simulink model "toa_wl00_sim"  (Simulink 9.0)
settings: Solver=FixedStepDiscrete  StartTime=0  StopTime=350  FixedStep=0.02  RelTol=1e-3  EnableMultiTasking=on
PreLoadFcn:
  | makefile_build_callback(bdroot,'toa_wl00.buildescription');
undefined symbols (not defined in the file or in its folder): TIME, timestep, WeighDebug_TOAarbitrated_payload, WeighDebug_TOAbucket_current_w_1, WeighDebug_TOAbucket_current_wei, WeighDebug_TOAcurrent_weight_nor, WeighDebug_TOAeef_imu_accelX, WeighDebug_TOAeef_imu_accelY, WeighDebug_TOAeef_imu_accelZ, WeighDebug_TOAerror_code_out, WeighDebug_TOAinvalidate_outputs, WeighDebug_TOAlift_angle, WeighDebug_TOAlift_he_pressure, WeighDebug_TOAlift_re_pressure, WeighDebug_TOAlift_valve_cmd, WeighDebug_TOApayload_norm_stdev, WeighDebug_TOApayload_send_to_CP, WeighDebug_TOApayload_status_sen, WeighDebug_TOApcs_weight_accurac, WeighDebug_TOAspill_rate_out, WeighDebug_TOAsteering_angle, WeighDebug_TOAtilt_extension, WeighDebug_TOAtilt_he_pressure, WeighDebug_TOAtilt_pressure_out, WeighDebug_TOAtilt_re_pressure, WeighDebug_TOAtilt_sensitivity_o, WeighDebug_TOAtilt_valve_cmd, WeighDebug_TOAtipoff_mode, WeighDebug_TOAtool_mass, WeighDebug_TOAtruck_start_weight, WeighDebug_TOAtruck_target_wt, WeighDebug_TOAweigh_status_out
libraries: simulink x30, lib_CATutils_Utilities_ApplyName_v2 x3, tip_assist_lib_support x1
settings Model: MinMaxOverflowLogging=MinMaxAndOverflow  Creator=gulamhs  LastModifiedBy=gulamhs  SimulationMode=accelerator
settings DataIOCC: ExternalInput=[t,u]  SaveCompleteFinalSimState=on  SaveFormat=StructureWithTime  SaveOutput=off  SignalLogging=off  DSMLogging=off  SaveTime=off
settings OptimizationCC: DefaultParameterBehavior=Inlined  InlineInvariantSignals=on  EnhancedBackFolding=on  StrengthReduction=on  BitfieldContainerType=uchar_T  PassReuseOutputArgsAs=Individual arguments  ExpressionDepthLimit=2147483647  EfficientFloat2IntCast=on
settings DebuggingCC: SignalInfNanChecking=warning  SignalRangeChecking=error  ReadBeforeWriteMsg=EnableAllAsError  WriteAfterWriteMsg=EnableAllAsError  WriteAfterReadMsg=EnableAllAsError  AlgebraicLoopMsg=error  ArtificialAlgebraicLoopMsg=error  SaveWithDisabledLinksMsg=error  SaveWithParameterizedLinksMsg=error  UnderspecifiedInitializationDetection=Simplified  MergeDetectMultiDrivingBlocksExec=error  BlockPriorityViolationMsg=error  SolverPrmCheckMsg=error  InheritedTsInSrcMsg=none  TasksWithSamePriorityMsg=error  SigSpecEnsureSampleTimeMsg=error  CheckMatrixSingularityMsg=error  IntegerOverflowMsg=error  ParameterUnderflowMsg=error  ParameterPrecisionLossMsg=none  FixptConstUnderflowMsg=error  FixptConstOverflowMsg=error  UnderSpecifiedDataTypeMsg=error  FcnCallInpInsideContextMsg=warning  UnconnectedInputMsg=error  UnconnectedOutputMsg=error  UnconnectedLineMsg=error  SFcnCompatibilityMsg=error  FrameProcessingCompatibilityMsg=warning  UniqueDataStoreMsg=error  BusObjectLabelMismatch=error  RootOutportRequireBusObject=error  AssertControl=DisableAll  ModelReferenceIOMsg=error  ModelReferenceVersionMismatchMessage=warning  ModelReferenceIOMismatchMessage=error  UnknownTsInhSupMsg=error  ModelReferenceDataLoggingMessage=error  StateNameClashWarn=warning  SimStateInterfaceChecksumMismatchMsg=error  StrictBusMsg=ErrorOnBusTreatedAsVector  BusNameAdapt=ErrorWithoutRepair  NonBusSignalsTreatedAsBus=error  SFInvalidInputDataAccessInChartInitDiag=error  SFNoUnconditionalDefaultTransitionDiag=error  SFTransitionOutsideNaturalParentDiag=error  SFUnreachableExecutionPathDiag=error  SFUndirectedBroadcastEventsDiag=error  SFExecutionAtInitializationDiag=warning  IntegerSaturationMsg=error
settings HardwareCC: ProdBitPerLong=64  ProdBitPerPointer=64  ProdBitPerSizeT=64  ProdBitPerPtrDiffT=64  ProdLargestAtomicInteger=Integer  ProdLargestAtomicFloat=Float  ProdIntDivRoundTo=Zero  ProdEndianess=LittleEndian  ProdWordSize=64  ProdHWDeviceType=Intel->x86-64 (Linux 64)
settings ModelReferenceCC: ParallelModelReferenceMATLABWorkerInit=Load Top Model  PropagateSignalLabelsOutOfModel=on
settings SFSimCC: SFSimEcho=off  SimGenImportedTypeDefs=on  MATLABDynamicMemAlloc=off
settings RTWCC: SystemTargetFile=cat_PkgArch.tlc  GenCodeOnly=on  GenerateMakefile=off  TemplateMakefile=cat_PkgArch_default_tmf  Description=R7a CAT Package Architecture Code Generation.  GenerateReport=on  RTWUseSimCustomCode=on  CodeProfilingSaveOptions=AllData  GenerateTraceReport=on  GenerateTraceReportSl=on  GenerateTraceReportSf=on  GenerateTraceReportEml=on  GenerateWebview=on  GenerateCodeMetricsReport=on  GenerateCodeReplacementReport=on
settings CodeAppCC: ForceParamTrailComments=on  IgnoreCustomStorageClasses=off  MaxIdLength=63  OperatorAnnotations=on  SimulinkDataObjDesc=on  SFDataObjDesc=on  MATLABFcnDesc=on  MangleLength=4  CustomSymbolStrType=$N$R$M  InsertBlockDesc=on  MATLABSourceComments=on  InternalIdentifier=Classic  ReqsInCode=on  UseSimReservedNames=on
settings STFCustomTargetCC: UtilityFuncGeneration=Shared location  MultiwordTypeDef=User defined  IncludeMdlTerminateFcn=off  CombineOutputUpdateFcns=on  SuppressErrorStatus=on  ERTCustomFileBanners=on  SupportAbsoluteTime=off  MultiInstanceERTCode=on  CodeInterfacePackaging=Reusable function  SupportComplex=off  SupportContinuousTime=off  SupportNonInlinedSFcns=off  RemoveResetFunc=on  SupportVariableSizeSignals=on  ParenthesesLevel=Maximum  MATLABClassNameForMDSCustomization=Simulink.SoftwareTarget.ERTCustomization  GRTInterface=off  GenerateSharedConstants=off  SystemTargetFile=cat_PkgArch.tlc
settings ERTTargetCC: UtilityFuncGeneration=Shared location  MultiwordTypeDef=User defined  MultiwordLength=2048  ParMdlRefBuildCompliant=off  CompOptLevelCompliant=off  ConcurrentExecutionCompliant=off  IncludeMdlTerminateFcn=off  SuppressErrorStatus=on  SupportAbsoluteTime=off  MultiInstanceERTCode=on  CodeInterfacePackaging=Reusable function  SupportComplex=off  SupportVariableSizeSignals=on  ParenthesesLevel=Maximum  ModelStepFunctionPrototypeControlCompliant=off  CPPClassGenCompliant=off  UseToolchainInfoCompliant=off  GenerateSharedConstants=off  MultiInstanceErrorCode=None  ERTSrcFileBannerTemplate=cat_code_template.cgt  ERTHdrFileBannerTemplate=cat_code_template.cgt  ERTDataSrcFileTemplate=cat_code_template.cgt  ERTDataHdrFileTemplate=cat_code_template.cgt  ERTCustomFileTemplate=cat_PkgArch_CFP.tlc  SuppressUnreachableDefaultCases=off  EnableUserReplacementTypes=on
settings MATStruct: int32=int32_t  int16=int16_t  int8=int8_t  uint32=uint32_t  uint16=uint16_t  uint8=uint8_t
settings CustomProperty: Value=Development
settings EnumStrPairs: String=Development
settings ConfigComp: CovMetricSettings=dwe  CovHtmlReporting=off  CovSaveCumulativeToWorkspaceVar=off  CovSaveSingleToWorkspaceVar=off  CovExternalEMLEnable=on

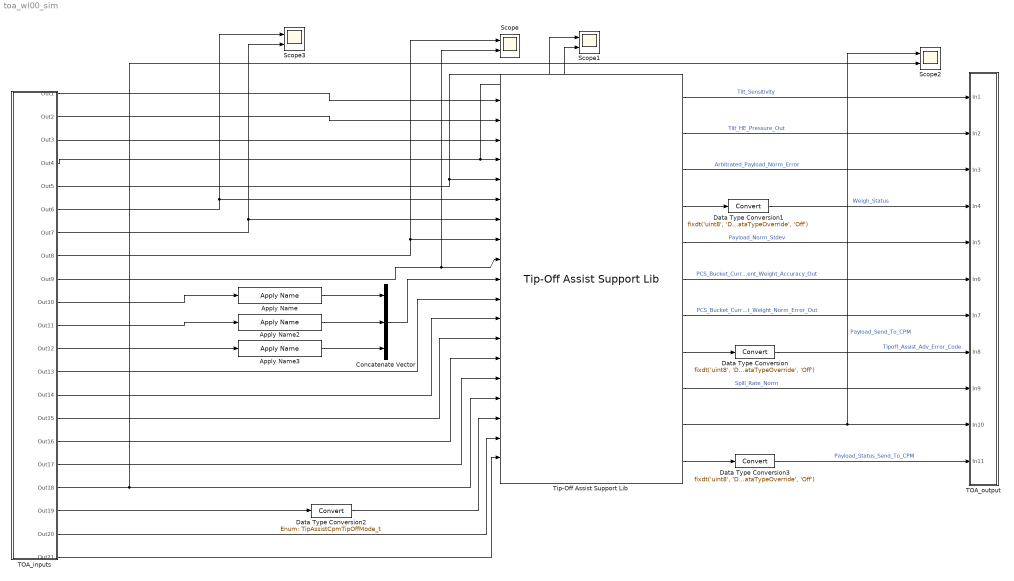
== system toa_wl00_sim ==
  Apply Name : lib_CATutils_Utilities_ApplyName_v2/Apply Name  sigLabel='toa_inImuAcclX'  enTst=true
  Apply Name2 : lib_CATutils_Utilities_ApplyName_v2/Apply Name  sigLabel='toa_inImuAcclY'  enTst=true
  Apply Name3 : lib_CATutils_Utilities_ApplyName_v2/Apply Name  sigLabel='toa_inImuAcclZ'  enTst=true
  Concatenate Vector : Concatenate  NumInputs=3  Mode=Multidimensional array
  Data Type Conversion : DataTypeConversion  OutMin=[0]  OutMax=[6]  OutDataTypeStr=fixdt('uint8', 'DataTypeOverride', 'Off')
  Data Type Conversion1 : DataTypeConversion  OutMin=[0]  OutMax=[5]  OutDataTypeStr=fixdt('uint8', 'DataTypeOverride', 'Off')
  Data Type Conversion2 : DataTypeConversion  OutDataTypeStr=Enum: TipAssistCpmTipOffMode_t
  Data Type Conversion3 : DataTypeConversion  OutMin=[0]  OutMax=[5]  OutDataTypeStr=fixdt('uint8', 'DataTypeOverride', 'Off')
  Scope{,1..3} (4 alike) : Scope  NumInputPorts=2
  "TOA_inputs " : Subsystem
  "TOA_output " : Subsystem
  Tip-Off Assist Support Lib : tip_assist_lib_support/Tip-Off Assist Support Lib
  wires:
  Apply Name2/1 -> Concatenate Vector/2
  Apply Name/1 -> Concatenate Vector/1
  Apply Name3/1 -> Concatenate Vector/3
  Concatenate Vector/1 -> Tip-Off Assist Support Lib/10
  Tip-Off Assist Support Lib/8 -> Data Type Conversion/1
  Tip-Off Assist Support Lib/4 -> Data Type Conversion1/1
  Data Type Conversion2/1 -> Tip-Off Assist Support Lib/17
  Tip-Off Assist Support Lib/11 -> Data Type Conversion3/1
  "TOA_inputs "/1(Out1) -> Tip-Off Assist Support Lib/1
  "TOA_inputs "/2(Out2) -> Tip-Off Assist Support Lib/2
  "TOA_inputs "/3(Out3) -> Tip-Off Assist Support Lib/3
  "TOA_inputs "/4(Out4) -> Tip-Off Assist Support Lib/4, Scope1/2
  "TOA_inputs "/5(Out5) -> Tip-Off Assist Support Lib/5, Scope1/1
  "TOA_inputs "/6(Out6) -> Tip-Off Assist Support Lib/6, Scope3/1
  "TOA_inputs "/7(Out7) -> Tip-Off Assist Support Lib/7, Scope3/2
  "TOA_inputs "/8(Out8) -> Tip-Off Assist Support Lib/8, Scope/1
  "TOA_inputs "/9(Out9) -> Scope/2, Tip-Off Assist Support Lib/9
  "TOA_inputs "/10(Out10) -> Apply Name/1
  "TOA_inputs "/11(Out11) -> Apply Name2/1
  "TOA_inputs "/12(Out12) -> Apply Name3/1
  "TOA_inputs "/13(Out13) -> Tip-Off Assist Support Lib/11
  Tip-Off Assist Support Lib/1 -> "TOA_output "/1(In1)  "Tilt_Sensitivity"
  Tip-Off Assist Support Lib/2 -> "TOA_output "/2(In2)  "Tilt_HE_Pressure_Out"
  Tip-Off Assist Support Lib/3 -> "TOA_output "/3(In3)  "Arbitrated_Payload_Norm_Error"
  Data Type Conversion1/1 -> "TOA_output "/4(In4)  "Weigh_Status"
  Tip-Off Assist Support Lib/5 -> "TOA_output "/5(In5)  "Payload_Norm_Stdev"
  Tip-Off Assist Support Lib/6 -> "TOA_output "/6(In6)  "PCS_Bucket_Current_Weight_Accuracy_Out"
  Tip-Off Assist Support Lib/7 -> "TOA_output "/7(In7)  "PCS_Bucket_Current_Weight_Norm_Error_Out"
  Data Type Conversion/1 -> "TOA_output "/8(In8)  "Tipoff_Assist_Adv_Error_Code"
  Tip-Off Assist Support Lib/9 -> "TOA_output "/9(In9)  "Spill_Rate_Norm"
  Tip-Off Assist Support Lib/10 -> Scope2/1, "TOA_output "/10(In10)  "Payload_Send_To_CPM"
  Data Type Conversion3/1 -> "TOA_output "/11(In11)  "Payload_Status_Send_To_CPM"
  "TOA_inputs "/14(Out14) -> Tip-Off Assist Support Lib/12
  "TOA_inputs "/15(Out15) -> Tip-Off Assist Support Lib/13
  "TOA_inputs "/16(Out16) -> Tip-Off Assist Support Lib/14
  "TOA_inputs "/17(Out17) -> Tip-Off Assist Support Lib/15
  "TOA_inputs "/18(Out18) -> Tip-Off Assist Support Lib/16, Scope2/2
  "TOA_inputs "/19(Out19) -> Data Type Conversion2/1
  "TOA_inputs "/20(Out20) -> Tip-Off Assist Support Lib/18
  "TOA_inputs "/21(Out21) -> Tip-Off Assist Support Lib/19

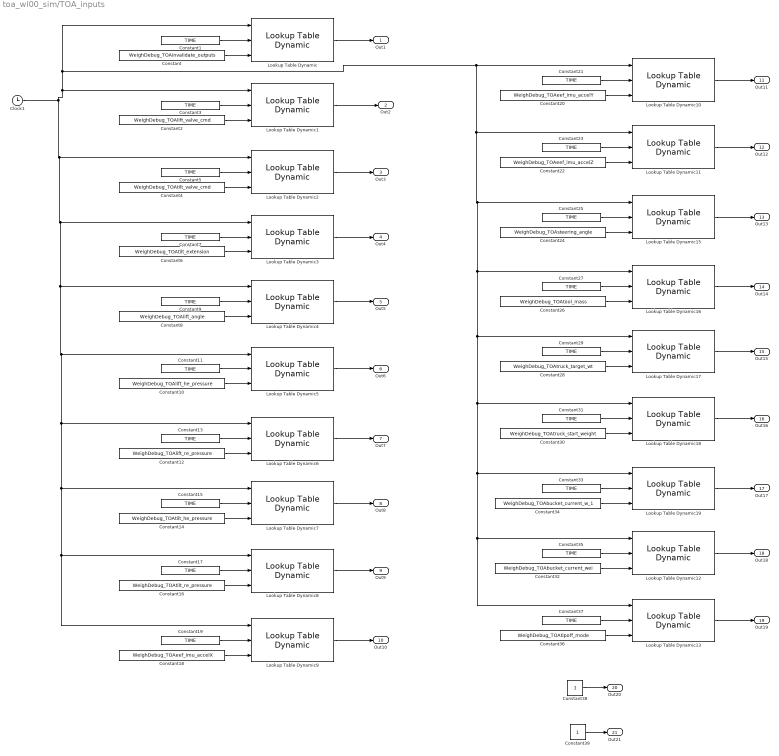
== system toa_wl00_sim/TOA_inputs  ==
  Clock1 : Clock
  Constant : Constant  Value=WeighDebug_TOAinvalidate_outputs  SampleTime=timestep
  Constant{1,3,5,7,9,11,13,15,17,19,21,23,25,27,29,31,33,35,37} (19 alike) : Constant  Value=TIME  SampleTime=timestep
  Constant10 : Constant  Value=WeighDebug_TOAlift_he_pressure  SampleTime=timestep
  Constant12 : Constant  Value=WeighDebug_TOAlift_re_pressure  SampleTime=timestep
  Constant14 : Constant  Value=WeighDebug_TOAtilt_he_pressure  SampleTime=timestep
  Constant16 : Constant  Value=WeighDebug_TOAtilt_re_pressure  SampleTime=timestep
  Constant18 : Constant  Value=WeighDebug_TOAeef_imu_accelX  SampleTime=timestep
  Constant2 : Constant  Value=WeighDebug_TOAlift_valve_cmd  SampleTime=timestep
  Constant20 : Constant  Value=WeighDebug_TOAeef_imu_accelY  SampleTime=timestep
  Constant22 : Constant  Value=WeighDebug_TOAeef_imu_accelZ  SampleTime=timestep
  Constant24 : Constant  Value=WeighDebug_TOAsteering_angle  SampleTime=timestep
  Constant26 : Constant  Value=WeighDebug_TOAtool_mass  SampleTime=timestep
  Constant28 : Constant  Value=WeighDebug_TOAtruck_target_wt  SampleTime=timestep
  Constant30 : Constant  Value=WeighDebug_TOAtruck_start_weight  SampleTime=timestep
  Constant32 : Constant  Value=WeighDebug_TOAbucket_current_wei  SampleTime=timestep
  Constant34 : Constant  Value=WeighDebug_TOAbucket_current_w_1  SampleTime=timestep
  Constant36 : Constant  Value=WeighDebug_TOAtipoff_mode  SampleTime=timestep
  Constant38 : Constant
  Constant39 : Constant
  Constant4 : Constant  Value=WeighDebug_TOAtilt_valve_cmd  SampleTime=timestep
  Constant6 : Constant  Value=WeighDebug_TOAtilt_extension  SampleTime=timestep
  Constant8 : Constant  Value=WeighDebug_TOAlift_angle  SampleTime=timestep
  Lookup Table Dynamic{,5..8,10..11,16..19} (11 alike) : simulink/Lookup Tables/Lookup Table Dynamic  LookUpMeth=Interpolation-Use End Values  OutDataType=fixdt('double')  OutScaling=2^-10  OutDataTypeStr=Inherit: Inherit via back propagation  DoSatur=off
      settings: SourceProductName=Simulink
  Lookup Table Dynamic{1..4,9,12,15} (7 alike) : simulink/Lookup Tables/Lookup Table Dynamic  LookUpMeth=Interpolation-Use End Values  OutDataType=fixdt('single')  OutScaling=[]  OutputDataTypeScalingMode=Specify via dialog  OutDataTypeStr=single  DoSatur=off
      settings: SourceProductName=Simulink
  Lookup Table Dynamic13 : simulink/Lookup Tables/Lookup Table Dynamic  LookUpMeth=Interpolation-Use End Values  OutDataType=fixdt('uint8')  OutScaling=[]  OutputDataTypeScalingMode=Specify via dialog  OutDataTypeStr=uint8  DoSatur=off
      settings: SourceProductName=Simulink
  Out1 : Outport  SampleTime=timestep
  Out2 : Outport  Port=2  SampleTime=timestep
  Out3 : Outport  Port=3  SampleTime=timestep
  Out4 : Outport  Port=4  SampleTime=timestep
  Out5 : Outport  Port=5  SampleTime=timestep
  Out6 : Outport  Port=6  SampleTime=timestep
  Out7 : Outport  Port=7  SampleTime=timestep
  Out8 : Outport  Port=8  SampleTime=timestep
  Out9 : Outport  Port=9  SampleTime=timestep
  Out10 : Outport  Port=10  SampleTime=timestep
  Out11 : Outport  Port=11  SampleTime=timestep
  Out12 : Outport  Port=12  SampleTime=timestep
  Out13 : Outport  Port=13  SampleTime=timestep
  Out14 : Outport  Port=14  SampleTime=timestep
  Out15 : Outport  Port=15  SampleTime=timestep
  Out16 : Outport  Port=16  SampleTime=timestep
  Out17 : Outport  Port=17  SampleTime=timestep
  Out18 : Outport  Port=18  SampleTime=timestep
  Out19 : Outport  Port=19  SampleTime=timestep
  Out20 : Outport  Port=20  SampleTime=timestep
  Out21 : Outport  Port=21  SampleTime=timestep
  wires:
  Constant17/1 -> Lookup Table Dynamic8/2
  Constant13/1 -> Lookup Table Dynamic6/2
  Lookup Table Dynamic6/1 -> Out7/1
  Lookup Table Dynamic5/1 -> Out6/1
  Constant/1 -> Lookup Table Dynamic/3
  Constant21/1 -> Lookup Table Dynamic10/2
  Lookup Table Dynamic2/1 -> Out3/1
  Constant3/1 -> Lookup Table Dynamic1/2
  Constant2/1 -> Lookup Table Dynamic1/3
  Lookup Table Dynamic9/1 -> Out10/1
  Constant8/1 -> Lookup Table Dynamic4/3
  Constant9/1 -> Lookup Table Dynamic4/2
  Constant12/1 -> Lookup Table Dynamic6/3
  Lookup Table Dynamic11/1 -> Out12/1
  Constant15/1 -> Lookup Table Dynamic7/2
  Lookup Table Dynamic7/1 -> Out8/1
  Lookup Table Dynamic8/1 -> Out9/1
  Constant16/1 -> Lookup Table Dynamic8/3
  Constant11/1 -> Lookup Table Dynamic5/2
  Constant14/1 -> Lookup Table Dynamic7/3
  Constant6/1 -> Lookup Table Dynamic3/3
  Constant23/1 -> Lookup Table Dynamic11/2
  Constant22/1 -> Lookup Table Dynamic11/3
  Lookup Table Dynamic/1 -> Out1/1
  Constant4/1 -> Lookup Table Dynamic2/3
  Lookup Table Dynamic3/1 -> Out4/1
  Lookup Table Dynamic4/1 -> Out5/1
  Constant1/1 -> Lookup Table Dynamic/2
  Constant18/1 -> Lookup Table Dynamic9/3
  Constant7/1 -> Lookup Table Dynamic3/2
  Constant20/1 -> Lookup Table Dynamic10/3
  Constant19/1 -> Lookup Table Dynamic9/2
  Lookup Table Dynamic10/1 -> Out11/1
  Constant5/1 -> Lookup Table Dynamic2/2
  Constant10/1 -> Lookup Table Dynamic5/3
  Lookup Table Dynamic1/1 -> Out2/1
  Constant32/1 -> Lookup Table Dynamic12/3
  Constant29/1 -> Lookup Table Dynamic17/2
  Constant36/1 -> Lookup Table Dynamic13/3
  Lookup Table Dynamic18/1 -> Out16/1
  Constant35/1 -> Lookup Table Dynamic12/2
  Lookup Table Dynamic16/1 -> Out14/1
  Constant24/1 -> Lookup Table Dynamic15/3
  Constant25/1 -> Lookup Table Dynamic15/2
  Constant27/1 -> Lookup Table Dynamic16/2
  Constant26/1 -> Lookup Table Dynamic16/3
  Lookup Table Dynamic19/1 -> Out17/1
  Lookup Table Dynamic15/1 -> Out13/1
  Lookup Table Dynamic13/1 -> Out19/1
  Constant34/1 -> Lookup Table Dynamic19/3
  Constant28/1 -> Lookup Table Dynamic17/3
  Lookup Table Dynamic17/1 -> Out15/1
  Constant30/1 -> Lookup Table Dynamic18/3
  Constant33/1 -> Lookup Table Dynamic19/2
  Constant37/1 -> Lookup Table Dynamic13/2
  Lookup Table Dynamic12/1 -> Out18/1
  Constant31/1 -> Lookup Table Dynamic18/2
  Clock1/1 -> Lookup Table Dynamic1/1, Lookup Table Dynamic13/1, Lookup Table Dynamic12/1, Lookup Table Dynamic19/1, Lookup Table Dynamic18/1, Lookup Table Dynamic17/1, Lookup Table Dynamic16/1, Lookup Table Dynamic15/1, Lookup Table Dynamic11/1, Lookup Table Dynamic10/1, Lookup Table Dynamic/1, Lookup Table Dynamic8/1, Lookup Table Dynamic9/1, Lookup Table Dynamic7/1, Lookup Table Dynamic6/1, Lookup Table Dynamic5/1, Lookup Table Dynamic4/1, Lookup Table Dynamic3/1, Lookup Table Dynamic2/1
  Constant38/1 -> Out20/1
  Constant39/1 -> Out21/1

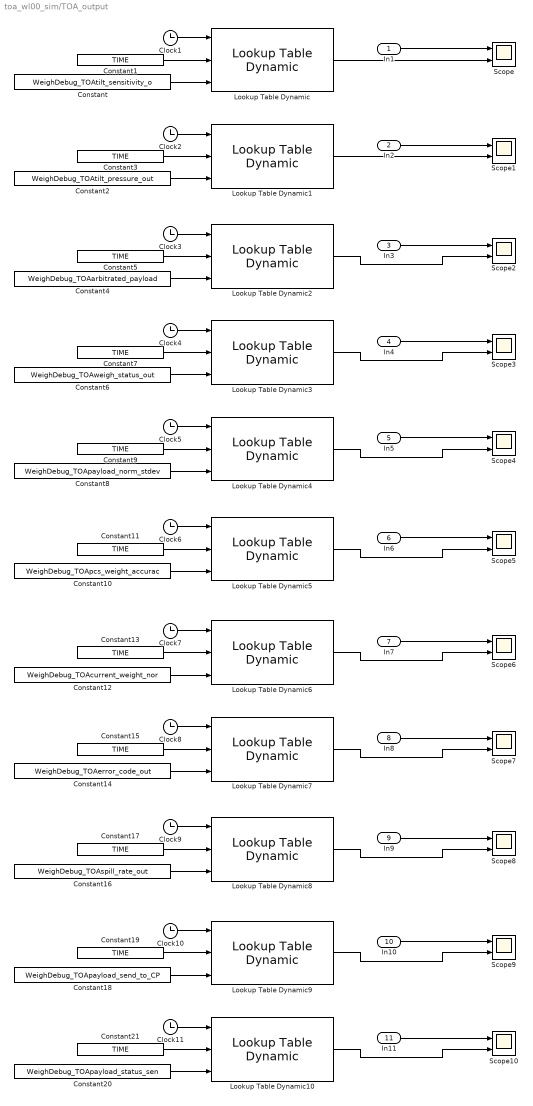
== system toa_wl00_sim/TOA_output  ==
  In1 : Inport
  In2 : Inport  Port=2
  In3 : Inport  Port=3
  In4 : Inport  Port=4
  In5 : Inport  Port=5
  In6 : Inport  Port=6
  In7 : Inport  Port=7
  In8 : Inport  Port=8
  In9 : Inport  Port=9
  In10 : Inport  Port=10
  In11 : Inport  Port=11
  Clock{1..11} (11 alike) : Clock
  Constant : Constant  Value=WeighDebug_TOAtilt_sensitivity_o  SampleTime=timestep
  Constant{1,3,5,7,9,11,13,15,17,19,21} (11 alike) : Constant  Value=TIME  SampleTime=timestep
  Constant10 : Constant  Value=WeighDebug_TOApcs_weight_accurac  SampleTime=timestep
  Constant12 : Constant  Value=WeighDebug_TOAcurrent_weight_nor  SampleTime=timestep
  Constant14 : Constant  Value=WeighDebug_TOAerror_code_out  SampleTime=timestep
  Constant16 : Constant  Value=WeighDebug_TOAspill_rate_out  SampleTime=timestep
  Constant18 : Constant  Value=WeighDebug_TOApayload_send_to_CP  SampleTime=timestep
  Constant2 : Constant  Value=WeighDebug_TOAtilt_pressure_out  SampleTime=timestep
  Constant20 : Constant  Value=WeighDebug_TOApayload_status_sen  SampleTime=timestep
  Constant4 : Constant  Value=WeighDebug_TOAarbitrated_payload  SampleTime=timestep
  Constant6 : Constant  Value=WeighDebug_TOAweigh_status_out  SampleTime=timestep
  Constant8 : Constant  Value=WeighDebug_TOApayload_norm_stdev  SampleTime=timestep
  Lookup Table Dynamic{,1..10} (11 alike) : simulink/Lookup Tables/Lookup Table Dynamic  LookUpMeth=Interpolation-Use End Values  OutDataType=fixdt('single')  OutScaling=[]  OutputDataTypeScalingMode=Specify via dialog  OutDataTypeStr=single  DoSatur=off
      settings: SourceProductName=Simulink
  Scope{,1..10} (11 alike) : Scope  NumInputPorts=2
  wires:
  Constant17/1 -> Lookup Table Dynamic8/2
  Clock8/1 -> Lookup Table Dynamic7/1
  Constant13/1 -> Lookup Table Dynamic6/2
  Clock4/1 -> Lookup Table Dynamic3/1
  Clock5/1 -> Lookup Table Dynamic4/1
  Constant/1 -> Lookup Table Dynamic/3
  Constant21/1 -> Lookup Table Dynamic10/2
  Constant3/1 -> Lookup Table Dynamic1/2
  Constant2/1 -> Lookup Table Dynamic1/3
  Clock1/1 -> Lookup Table Dynamic/1
  Constant8/1 -> Lookup Table Dynamic4/3
  Constant9/1 -> Lookup Table Dynamic4/2
  Constant12/1 -> Lookup Table Dynamic6/3
  Constant15/1 -> Lookup Table Dynamic7/2
  Clock3/1 -> Lookup Table Dynamic2/1
  Constant16/1 -> Lookup Table Dynamic8/3
  Constant11/1 -> Lookup Table Dynamic5/2
  Constant14/1 -> Lookup Table Dynamic7/3
  Clock7/1 -> Lookup Table Dynamic6/1
  Constant6/1 -> Lookup Table Dynamic3/3
  Clock2/1 -> Lookup Table Dynamic1/1
  Clock6/1 -> Lookup Table Dynamic5/1
  Lookup Table Dynamic/1 -> Scope/2
  Constant4/1 -> Lookup Table Dynamic2/3
  Clock9/1 -> Lookup Table Dynamic8/1
  Constant1/1 -> Lookup Table Dynamic/2
  Clock10/1 -> Lookup Table Dynamic9/1
  Constant18/1 -> Lookup Table Dynamic9/3
  Constant7/1 -> Lookup Table Dynamic3/2
  Clock11/1 -> Lookup Table Dynamic10/1
  Constant20/1 -> Lookup Table Dynamic10/3
  Constant19/1 -> Lookup Table Dynamic9/2
  Constant5/1 -> Lookup Table Dynamic2/2
  Constant10/1 -> Lookup Table Dynamic5/3
  In1/1 -> Scope/1
  In2/1 -> Scope1/1
  Lookup Table Dynamic1/1 -> Scope1/2
  In3/1 -> Scope2/1
  Lookup Table Dynamic2/1 -> Scope2/2
  In4/1 -> Scope3/1
  Lookup Table Dynamic3/1 -> Scope3/2
  In5/1 -> Scope4/1
  Lookup Table Dynamic4/1 -> Scope4/2
  In6/1 -> Scope5/1
  Lookup Table Dynamic5/1 -> Scope5/2
  In7/1 -> Scope6/1
  Lookup Table Dynamic6/1 -> Scope6/2
  In8/1 -> Scope7/1
  Lookup Table Dynamic7/1 -> Scope7/2
  In9/1 -> Scope8/1
  Lookup Table Dynamic8/1 -> Scope8/2
  In10/1 -> Scope9/1
  Lookup Table Dynamic9/1 -> Scope9/2
  In11/1 -> Scope10/1
  Lookup Table Dynamic10/1 -> Scope10/2
